simulink model "pcssp_controller_and_ps"  (R2024b)
settings: Solver=VariableStepAuto  StartTime=t_start  StopTime=t_max  RelTol=1e-3
values from neighbouring files (symbols this model uses):
  AllocatorMode = 1    [muscle_controller_NICE_IMAS_iter_init.m]
  enable_KCURR = double(instance.get_setting('KCURR', pyargs('default', 1)))    [muscle_controller_NICE_IMAS_iter_init.m]
  enable_RZIp = double(instance.get_setting('RZIp', pyargs('default', 0)))    [muscle_controller_NICE_IMAS_iter_init.m]
  enable_VS = double(instance.get_setting('VS', pyargs('default', 1)))    [muscle_controller_NICE_IMAS_iter_init.m]
  in_out_dt = double(instance.get_setting('in_out_msg_dt', pyargs('default', 0.001)))    [muscle_controller_NICE_IMAS_iter_init.m]
  IpControlMode = 0    [muscle_controller_NICE_IMAS_iter_init.m]
  IpControlMode_KCURR = double(instance.get_setting('control_Ip', pyargs('default', 1)))    [muscle_controller_NICE_IMAS_iter_init.m]
  IpControlMode_RZIp = 0    [muscle_controller_NICE_IMAS_iter_init.m]
  RZIp_R_sign = double(instance.get_setting('RZIp_R_sign', pyargs('default', sign(mean(ip_ref)) + (mean(ip_ref) == 0))))    [muscle_controller_NICE_IMAS_iter_init.m]
  RZIp_Z_sign = double(instance.get_setting('RZIp_Z_sign', pyargs('default', RZIp_R_sign)))    [muscle_controller_NICE_IMAS_iter_init.m]
  schedulingVar_KCURR = 0    [muscle_controller_NICE_IMAS_iter_init.m]
  SchedulingVar_ShapeContr = VSControlMode    [muscle_controller_NICE_IMAS_iter_init.m]
  SCIpScaling = double(instance.get_setting('SC_Ip_scaling', pyargs('default', 1)))    [muscle_controller_NICE_IMAS_iter_init.m]
  ShapeIpControlMode = double(instance.get_setting('shape_control', pyargs('default', 0)))    [muscle_controller_NICE_IMAS_iter_init.m]
  usePSModel = double(instance.get_setting('PSModel', pyargs('default', 1)))    [muscle_controller_NICE_IMAS_iter_init.m]
  VSControlMode = double(instance.get_setting('VS_control_mode', pyargs('default', 3)))    [muscle_controller_NICE_IMAS_iter_init.m]
  VSIpScaling = 1    [muscle_controller_NICE_IMAS_iter_init.m]
Description:
  | The KCURR_PFPO1 module implements a CS/PF current controller, including control of IpThis version performs internal gain scheduling based on an externally fed scheduling variable. Note: the coils are sorted as CS3U CS2U CS1 CS2L CS3L P1 P2 P3 P4 P5 P6
settings Model: VariantFading=off  Creator=ravenst1  LastModifiedBy=schneim
settings SolverCC: AutoInsertRateTranBlk=on
settings DebuggingCC: UnderspecifiedInitializationDetection=Classic  MergeDetectMultiDrivingBlocksExec=none
settings ModelReferenceCC: PropagateSignalLabelsOutOfModel=off

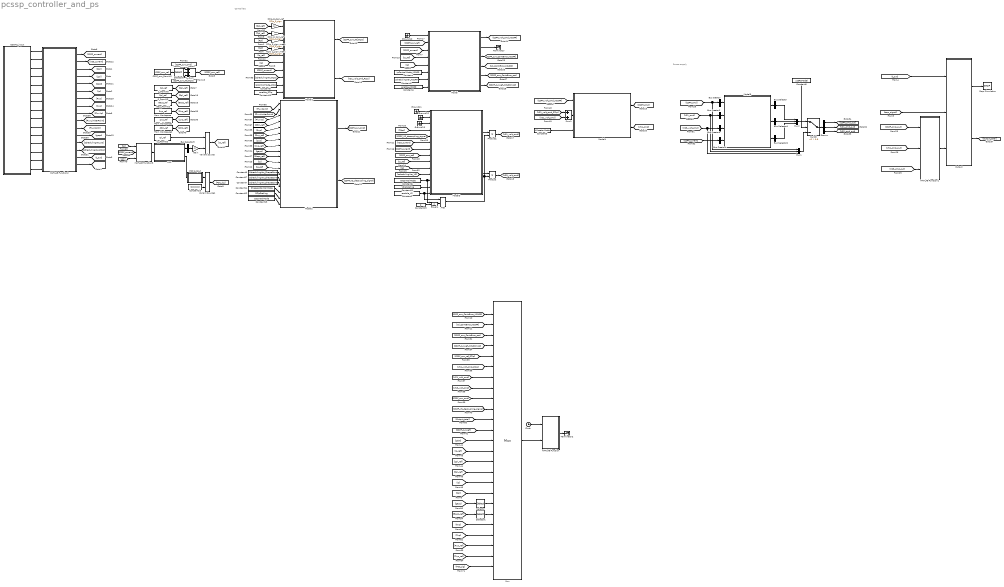
== system pcssp_controller_and_ps ==
  note: Power supply
  note: Controllers
  AND : Logic  IconShape=distinctive  AllPortsSameDT=off  OutDataTypeStr=boolean
  Bus Creator : BusCreator  Inputs=1  OutDataTypeStr=Bus:pcssp_PS_CSPF_volt_cmd
  Bus Creator2 : BusCreator  Inputs=1  OutDataTypeStr=Bus: pcssp_PS_VS1_volt_cmd
  Bus Creator3 : BusCreator  Inputs=1  OutDataTypeStr=Bus: pcssp_PS_VS3_volt_cmd
  Bus Creator4 : BusCreator  Inputs=1  OutDataTypeStr=Bus: pcssp_PS_CSPF_curr_meas
  Bus Selector : BusSelector  OutputSignals=VCSPF
  Bus Selector1 : BusSelector  OutputSignals=VS1
  Bus Selector2 : BusSelector  OutputSignals=VS3
  Bus Selector3 : BusSelector  OutputSignals=psc_ref__Ipl_ref
  CODAC_input : MATLAB Function  TreatAsAtomicUnit=on  SystemSampleTime=in_out_dt
  CSPF_curr_FromWS : FromWorkspace  VariableName=CSPF_curr_ref
  Clock : Clock
  Constant : Constant  Value=IpControlMode_KCURR  OutDataTypeStr=boolean
  Constant1 : Constant  Value=schedulingVar_KCURR
  Constant10 : Constant  Value=enable_RZIp  OutDataTypeStr=boolean
  Constant11 : Constant  Value=VSIpScaling
  Constant12 : Constant  Value=SCIpScaling
  Constant13 : Constant  Value=IpControlMode
  Constant14 : Constant  Value=ShapeIpControlMode
  Constant15 : Constant  Value=0
  Constant16 : Constant  Value=[0;0;0;0]
  Constant17 : Constant  Value=SchedulingVar_ShapeContr
  Constant2 : Constant  Value=enable_VS  OutDataTypeStr=boolean
  Constant3 : Constant  Value=AllocatorMode
  Constant4 : Constant  Value=enable_KCURR
  Constant5 : Constant  Value=usePSModel
  Constant6 : Constant  Value=VSControlMode
  Constant7 : Constant  Value=SchedulingVar_ShapeContr
  Constant8 : Constant  Value=IpControlMode_RZIp  OutDataTypeStr=boolean
  Constant9 : Constant  Value=SchedulingVar_ShapeContr
  Demux : Demux  Outputs=[11 1 1]
  Equal4 : RelationalOperator  Operator=>  OutDataTypeStr=boolean  RndMeth=Simplest  InputSameDT=off
  From Workspace : FromWorkspace  VariableName=Rxp_ref
  From Workspace1 : FromWorkspace  VariableName=Zxp_ref
  From Workspace2 : FromWorkspace  VariableName=dPsi_ref
  Gain : Gain  Gain=-1
  Gap_FromWS : FromWorkspace  VariableName=Gaps_ref
  Ground{10..13} (4 alike) : Ground
  Ip_FromWS : FromWorkspace  VariableName=Ipl_ref
  MATLAB Function : MATLAB Function  TreatAsAtomicUnit=on  SystemSampleTime=in_out_dt
  MATLAB Function1 : MATLAB Function  TreatAsAtomicUnit=on  SystemSampleTime=in_out_dt
  MATLAB Function2 : MATLAB Function  TreatAsAtomicUnit=on  SystemSampleTime=in_out_dt
  MATLAB Function3 : MATLAB Function  TreatAsAtomicUnit=on
  Model : ModelReference  ModelNameDialog=pcssp_KCURR_PFPO1.slx  SimulationMode=Normal  ModelReferenceVersion=6.1
  Model1 : ModelReference  ModelNameDialog=pcssp_RZIp_CCS.slx  SimulationMode=Normal  ModelReferenceVersion=10.5
  Model2 : ModelReference  ModelNameDialog=shapeIp_CCS.slx  SimulationMode=Normal  ModelReferenceVersion=1.1
  Model3 : ModelReference  ModelNameDialog=pcssp_VS.slx  SimulationMode=Normal  ModelReferenceVersion=7.2
  Model4 : ModelReference  ModelNameDialog=VS1_allocator.slx  SimulationMode=Normal  ModelReferenceVersion=1.4
  Model5 : ModelReference  ModelNameDialog=pcssp_PowerSupplies.slx  ParameterArgumentNames=PS_tp  UsingDefaultArgumentValue=0  SimulationMode=Normal  ModelReferenceVersion=1.39
  Mux : Mux  Inputs=25
      settings: DisplayOption=signals
  Mux1 : Mux  Inputs=3
  Mux2 : Mux  Inputs=3
  Output : MATLAB Function  TreatAsAtomicUnit=on  SystemSampleTime=in_out_dt
  PSC : Subsystem  ReferencedSubsystem=PSC  ConfFolderPath=/home/ITER/centong/Desktop/PDSs/IMAS-PDS-torax/cases/input/psc/A_nom/psc_config_ip_105073_psc_A_nom  PSCInterConfFileName=BTree.xml  GlobMonFileName=BTree.xml  DecisionFileName=BTree.xml  RefGenFileName=BTree.xml  useInBus=Bus signal  useInPorts=Ports  useOutBus=Bus signal  useOutPorts=Ports  SaveStatus=off
  PSC output : MATLAB Function  TreatAsAtomicUnit=on
  Product : Product
  Product1 : Product
  RZIp_R_sign_meas : Gain  Gain=RZIp_R_sign
  RZIp_R_sign_ref : Gain  Gain=RZIp_R_sign
  RZIp_Z_sign_meas : Gain  Gain=RZIp_Z_sign
  RZIp_Z_sign_ref : Gain  Gain=RZIp_Z_sign
  R_FromWS : FromWorkspace  VariableName=Rpl_ref
  Selector : Selector  InputPortWidth=N_GAPS  IndexOptions=Index vector (dialog)  Indices=GAP_LIST  OutputSizes=1
  Selector1 : Selector  InputPortWidth=N_GAPS  IndexOptions=Index vector (dialog)  Indices=GAP_LIST  OutputSizes=1
  Selector3 : Selector  IndexMode=Zero-based  InputPortWidth=14  IndexOptions=Index vector (dialog)  Indices=[0 1 2 4 5 6 7 8 9 10 11]  OutputSizes=1
  Stop Simulation : Stop
  Sum : Sum  Inputs=+++
  Sum1 : Sum
  Switch : Switch  Criteria=u2 > Threshold  Threshold=0.5  SaturateOnIntegerOverflow=off  InputSameDT=off
  Terminator : Terminator
  Terminator2 : Terminator
  Variant Source : VariantSource
  Variant Source1 : VariantSource
  Z_FromWS : FromWorkspace  VariableName=Zpl_ref
  wires:
  CODAC_input/1(coils_current) -> MATLAB Function2/1(coil_currents)  "current_coils"
  Model/1 -> [CSPF_volt_cmd_KCURR]
  Constant1/1 -> Model/7
  Constant/1 -> Model/6
  Constant8/1 -> Model1/9
  [schedulingVar_RZIp] -> Model1/8
  CSPF_curr_FromWS/1 -> Selector3/1
  Model/2 -> Terminator/1
  Model1/1 -> [CSPF_curr_ref_RZIp]
  Output/1(stop_signal_out) -> Stop Simulation/1
  [Ip] -> Model/5
  [t_out] -> Output/1(t_cur)
  [stop_signal] -> Output/2(stop_signal)
  [CSPF_current] -> Model/3
  [CSPF_current] -> Model1/7
  Z_FromWS/1 -> [Zpl_ref]
  Ground11/1 -> Model3/1
  [Ip_ref] -> Model/4
  [schedulingVar_VS] -> Model3/11
  Constant6/1 -> Equal4/1, Model3/12
  [CSPF_curr_ref] -> Model/2
  [Zdot] -> Model3/4
  Constant11/1 -> Model3/13
  Gap_FromWS/1 -> [Gaps_ref]
  Model1/2 -> [VS1_volt_cmd_RZIp]
  Equal4/1 -> AND/2
  Constant15/1 -> Equal4/2
  Model3/2 -> Product/1
  Product/1 -> [VS3_volt_cmd]
  AND/1 -> Product1/2, Product/2
  Product1/1 -> [VS1_volt_cmd]
  Model3/1 -> Product1/1
  R_FromWS/1 -> [Rpl_ref]
  [CSPF_current] -> Model3/7
  [VS3_current] -> Model3/6
  [CSPF_curr_ref] -> Model3/8
  Model2/1 -> [CSPF_curr_cmd]
  [CSPF_curr_cmd] -> Sum/1
  [CSPF_curr_ref_RZIp] -> Sum/3
  Sum/1 -> [CSPF_curr_ref]
  [Ip_ref] -> Model2/12
  [gaps] -> Model2/9
  [Rxp_ref] -> Model2/6
  Constant7/1 -> Model2/15
  Constant17/1 -> Model2/14
  [Ip] -> Model2/11
  [Gaps_ref] -> Model2/10
  [dPsi_ref] -> Model2/4
  Constant12/1 -> Model2/17
  Constant9/1 -> Model2/13
  [FluxContr] -> Model2/1
  Model2/2 -> [CSPF_VS_decoupling_signal]
  [Zxp_ref] -> Model2/8
  [FluxXp] -> Model2/3
  [Zxp] -> Model2/7
  [Rxp] -> Model2/5
  Constant14/1 -> Model2/16
  [CSPF_VS_decoupling_signal] -> Model3/5
  Model/6 -> [CSPF_curr_ref_KCURRmod]
  Model/5 -> [CSPF_curr_ContrError_res]
  Model/4 -> [Ipl_ContrError_KCURR]
  Model/3 -> [CSPF_curr_ContrError_KCURR]
  Constant10/1 -> Model1/10
  Constant4/1 -> Model/8
  Constant2/1 -> AND/1, Model3/14
  Constant13/1 -> Model2/18
  [Ip_ref] -> Model3/9
  [Ip] -> Model3/10
  [Ip_ref] -> Model1/5
  [Ip] -> Model1/6
  Ground10/1 -> Model/1
  Ground12/1 -> Model3/2
  Ground13/1 -> Model3/3
  Ip_FromWS/1 -> Variant Source/1
  Selector3/1 -> Sum/2
  [CSPF_volt_cmd_KCURR] -> Model4/1
  [VS1_volt_cmd_RZIp] -> Sum1/1
  [VS1_volt_cmd] -> Sum1/2
  Sum1/1 -> Model4/2
  Model4/2 -> [VS1_cmd]
  Model4/1 -> [CSPF_cmd]
  Constant3/1 -> Model4/3
  CODAC_input/2(rpl) -> MATLAB Function2/2(rpl)  "rgeo"
  CODAC_input/3(zpl) -> MATLAB Function2/3(zpl)  "zgeo"
  CODAC_input/5(ip) -> MATLAB Function2/5(ip)  "ip"
  CODAC_input/11(gaps) -> MATLAB Function2/11(gaps)
  CODAC_input/12(li3) -> MATLAB Function2/12(li3)
  CODAC_input/13(schedulingVar_RZIp) -> MATLAB Function2/13(schedulingVar_RZIp)
  CODAC_input/14(t_out) -> MATLAB Function2/14("t ")  "t_msg"
  MATLAB Function2/1(Icspf_meas) -> [CSPF_current]
  MATLAB Function2/2(Ivs3_meas) -> [VS3_current]
  MATLAB Function2/3(rpl_meas) -> [Rpl]
  MATLAB Function2/4(zpl_meas) -> [Zpl]
  MATLAB Function2/5(zdot_meas) -> [Zdot]
  MATLAB Function2/6(ip_meas) -> [Ip]
  MATLAB Function2/12(gaps_meas) -> [gaps]
  MATLAB Function2/14(sched_meas) -> [schedulingVar_RZIp]
  MATLAB Function2/13(li3_meas) -> [schedulingVar_VS]
  MATLAB Function1/1(total_cmd) -> Output/3("voltage ")
  [CSPF_cmd_out] -> MATLAB Function1/1(cspfout)
  [VS1_cmd_out] -> MATLAB Function1/2(vs1out)
  [VS3_cmd_out] -> MATLAB Function1/3(vs3out)
  [CSPF_cmd] -> Mux1/1, Bus Creator/1  "CSPF_volt_cmd"
  Bus Creator/1 -> Model5/1
  Bus Creator2/1 -> Model5/2
  [VS1_cmd] -> Mux1/2, Bus Creator2/1  "VS1_volt_cmd"
  [VS3_volt_cmd] -> Mux1/3, Bus Creator3/1  "VS3_volt_cmd"
  Bus Creator3/1 -> Model5/3
  [CSPF_current] -> Bus Creator4/1  "CSPF_curr_meas"
  Bus Creator4/1 -> Model5/4
  Model5/1 -> Bus Selector/1
  Bus Selector/1 -> Mux2/1  "<VCSPF>"
  Bus Selector1/1 -> Mux2/2  "<VS1>"
  Model5/2 -> Bus Selector1/1
  Model5/3 -> Bus Selector2/1
  Bus Selector2/1 -> Mux2/3  "<VS3>"
  Mux2/1 -> Switch/1
  Mux1/1 -> Switch/3
  Constant5/1 -> Switch/2
  Switch/1 -> Demux/1
  Demux/1 -> [CSPF_cmd_out]
  Demux/2 -> [VS1_cmd_out]
  Demux/3 -> [VS3_cmd_out]
  CODAC_input/6(r_xp) -> MATLAB Function2/6(r_xp)
  CODAC_input/7(z_xp) -> MATLAB Function2/7(z_xp)
  CODAC_input/8(psi_xp) -> MATLAB Function2/8(psi_xp)
  [VS1_volt_cmd] -> Mux/7  "VS_VS1_cmd"
  [CSPF_curr_ref_KCURRmod] -> Mux/4  "KCURR_actual_ref"
  [Ip] -> Mux/17
  [Gaps_ref] -> Selector1/1
  MATLAB Function/1(y) -> Terminator2/1
  Selector1/1 -> Mux/20  "gaps_ref"
  [Rpl_ref] -> Mux/16  "R_ref"
  [Ip_ref] -> Mux/14  "Ip_ref"
  Selector/1 -> Mux/19  "gaps"
  [CSPF_curr_ref_RZIp] -> Mux/5  "RZIp_CSPF_curr_cmd"
  [VS1_volt_cmd_RZIp] -> Mux/6  "RZIp_VS1_cmd"
  [Zdot] -> Mux/13  "Z_dot"
  [CSPF_curr_ContrError_res] -> Mux/3  "KCURR_residual_ctrl_e"
  [CSPF_curr_cmd] -> Mux/9  "Shape_CSPF_curr_cmd"
  [VS3_volt_cmd] -> Mux/8  "VS_VS3_cmd"
  [CSPF_VS_decoupling_signal] -> Mux/10  "Shape_VS_decoupling"
  [CSPF_curr_ref] -> Mux/12  "CSPF_curr_ref"
  [gaps] -> Selector/1
  [CSPF_curr_ContrError_KCURR] -> Mux/1  "KCURR_CSPF_ctrl_e"
  [Zpl] -> Mux/18
  Clock/1 -> MATLAB Function/1(t)
  [Zpl_ref] -> Mux/15  "Z_ref"
  [Ipl_ContrError_KCURR] -> Mux/2  "KCURR_Ip_ctrl_e"
  Mux/1 -> MATLAB Function/2(u)
  MATLAB Function2/7(rxp_meas) -> [Rxp]
  MATLAB Function2/8(zxp_meas) -> [Zxp]
  MATLAB Function2/9(psixp_meas) -> [FluxXp]
  From Workspace/1 -> [Rxp_ref]
  From Workspace1/1 -> [Zxp_ref]
  Output/2(voltage) -> [Output_total]  "Output_total"
  [Output_total] -> Mux/11
  MATLAB Function2/15(t) -> [t_out]
  CODAC_input/15(stop_signal) -> MATLAB Function2/15("stop_signal ")
  MATLAB Function2/16(stop_signal) -> [stop_signal]
  [Rxp] -> Mux/21
  [Zxp] -> Mux/22
  [Rxp_ref] -> Mux/23  "Rxp_ref"
  [Zxp_ref] -> Mux/24  "Zxp_ref"
  CODAC_input/9(PsiLimiter) -> MATLAB Function2/9(PsiLimiter)
  MATLAB Function2/10(psiLimiter_meas) -> [FluxLimiterPoint]
  [FluxLimiterPoint] -> Model2/2
  CODAC_input/10(flux_contr) -> MATLAB Function2/10(flux_contr)
  MATLAB Function2/11(fluxCtrl_meas) -> [FluxContr]
  From Workspace2/1 -> [dPsi_ref]
  CODAC_input/4(zdot) -> MATLAB Function2/4(zdot)
  MATLAB Function3/1(inb) -> PSC/1
  PSC/1 -> Bus Selector3/1
  Bus Selector3/1 -> Gain/1  "<psc_ref__Ipl_ref>"
  Variant Source/1 -> [Ip_ref]
  Gain/1 -> Variant Source/2
  [Ip] -> MATLAB Function3/1(ip)
  [CSPF_current] -> MATLAB Function3/2(Icspf)
  [Zpl] -> MATLAB Function3/3(z)
  PSC/2 -> PSC output/1(intb)
  Constant16/1 -> Variant Source1/2
  PSC output/1(y) -> Variant Source1/1
  Variant Source1/1 -> [PSC_sig]
  [PSC_sig] -> Mux/25  "PSC_sig"
  [Rpl_ref] -> RZIp_R_sign_ref/1
  RZIp_R_sign_ref/1 -> Model1/1
  [Zpl_ref] -> RZIp_Z_sign_ref/1
  RZIp_Z_sign_ref/1 -> Model1/2
  [Rpl] -> RZIp_R_sign_meas/1
  RZIp_R_sign_meas/1 -> Model1/3
  [Zpl] -> RZIp_Z_sign_meas/1
  RZIp_Z_sign_meas/1 -> Model1/4

== matlab function pcssp_controller_and_ps/MATLAB Function ==
  data: t input; u input; y output
function y = csv_logger(t,u)
coder.extrinsic('log_row');
log_row(t, u);
y = 0;
end

== matlab function pcssp_controller_and_ps/MATLAB Function3 ==
  data: ip input; inb output Bus: PSC_In_Bus; Icspf input; z input
function inb = psc_input(ip, Icspf, z)
% PSC_In_Bus from the measurements (PCS frame: Ip > 0)
inb.ip_ip__meas.value = -ip;
inb.ip_ip__meas.quality = PcsQuality_t.kGood;
inb.ip_ip__meas.activity = PcsActivity_t.kRunning;
inb.plasma_state__exist_diag.value = 1;
inb.plasma_state__exist_diag.quality = PcsQuality_t.kGood;
inb.plasma_state__exist_diag.activity = PcsActivity_t.kRunning;
inb.z_meas.value = z;
inb.z_meas.quality = PcsQuality_t.kGood;
inb.z_meas.activity = PcsActivity_t.kRunning;
inb.cs_margin.value = min(45e3 - abs(Icspf(1:5)));  
inb.cs_margin.quality = PcsQuality_t.kGood;
inb.cs_margin.activity = PcsActivity_t.kRunning;
end

== matlab function pcssp_controller_and_ps/Output ==
  data: t_cur input; stop_signal input; voltage input; stop_signal_out output; voltage output
function [stop_signal_out, voltage] = CODAC_output(t_cur, stop_signal,voltage)



% constrain python function to run extrinsically in Matlab (no codegen)
coder.extrinsic('muscle_control2nice');

muscle_control2nice(t_cur,voltage);

stop_signal_out = stop_signal;

== matlab function pcssp_controller_and_ps/PSC output ==
  data: intb input Bus: PSC_Int_Bus; y output
function y = psc_output(intb)
y = [intb.psc_ref__current_segment; double(intb.glb_ps__ip_too_high); ...
     double(intb.glb_ps__end_of_flux); double(intb.glb_ps__z_excursion)];
end

== matlab function pcssp_controller_and_ps/CODAC_input ==
  data: coils_current output; rpl output; zpl output; zdot output; ip output; r_xp output; z_xp output; psi_xp output; PsiLimiter output; flux_contr output; gaps output; li3 output; schedulingVar_RZIp output; t_out output; stop_signal output
function [coils_current,rpl,zpl,zdot,ip,r_xp,z_xp,psi_xp,PsiLimiter,flux_contr,gaps,li3,schedulingVar_RZIp,t_out,stop_signal]  = CODAC_input
% Receives the plant measurements from MUSCLE3 (muscle_nice2control, run in MATLAB).

% outputs of an extrinsic call: size and type must be declared beforehand
N_GAPS = 62;
coils_current = zeros(14,1);
rpl = 0;
zpl = 0;
ip = 0;
gaps = zeros(N_GAPS,1);
li3 = 0;
zdot = 0;
schedulingVar_RZIp = zeros(3,1);
flux_contr = zeros(62,1);
r_xp = 0;
z_xp = 0;
psi_xp = 0;
PsiLimiter = 0;
t_out = 0;
stop_signal = 0;

% runs in MATLAB, not compiled (it calls MUSCLE3 through Python)
coder.extrinsic('muscle_nice2control');

[coils_current,rpl,zpl,zdot,ip,r_xp,z_xp,psi_xp,PsiLimiter,flux_contr,gaps,li3,schedulingVar_RZIp,t_out,stop_signal] = muscle_nice2control();
end

== matlab function pcssp_controller_and_ps/MATLAB Function1 ==
  data: cspfout input; total_cmd output; vs1out input; vs3out input
function total_cmd = output_block(cspfout, vs1out, vs3out)
    coder.extrinsic('controller_output_preprocess');
    total_cmd = zeros(14,1);
    total_cmd = controller_output_preprocess(cspfout, vs1out, vs3out);
end

== matlab function pcssp_controller_and_ps/MATLAB Function2 ==
  data: coil_currents input; Icspf_meas output; rpl input; zpl input; zdot input; ip input; r_xp input; z_xp input; psi_xp input; PsiLimiter input; flux_contr input; gaps input; li3 input; schedulingVar_RZIp input; t input; Ivs3_meas output; rpl_meas output; zpl_meas output; zdot_meas output; ip_meas output; rxp_meas output; zxp_meas output; psixp_meas output; psiLimiter_meas output; fluxCtrl_meas output; gaps_meas output; li3_meas output; sched_meas output; t output; stop_signal input; stop_signal output
function [Icspf_meas,Ivs3_meas,rpl_meas,zpl_meas,zdot_meas,ip_meas,rxp_meas,zxp_meas,psixp_meas,psiLimiter_meas,fluxCtrl_meas,gaps_meas,li3_meas,sched_meas,t,stop_signal] = preprocess_block(coil_currents,rpl,zpl,zdot, ip,r_xp,z_xp,psi_xp,PsiLimiter, flux_contr, gaps,li3,schedulingVar_RZIp,t,stop_signal)

coder.extrinsic('controller_input_preprocess');

% declare size
Icspf_meas = zeros(11,1);
Ivs3_meas  = 0;
zdot_meas = 0;

[Icspf_meas,Ivs3_meas,zdot_meas] = controller_input_preprocess(coil_currents,ip,zdot,t);

% no preprocessing: passed through
rpl_meas = rpl;
zpl_meas = zpl;
ip_meas = ip;
rxp_meas = r_xp;
zxp_meas = z_xp;
psixp_meas = psi_xp;
psiLimiter_meas = PsiLimiter;
gaps_meas = gaps;
li3_meas = li3;
sched_meas = schedulingVar_RZIp;
fluxCtrl_meas = flux_contr;
end
